simulink model "AGV_Warehouse_Sim_backup_before_v2"  (R2024b)
settings: Solver=ode23t  StartTime=0.0  StopTime=90  MaxStep=0.005  RelTol=1e-3
model workspace: external: MATLAB File D:\agv_robot_matlab\AGV_DataFile.m (data not in the file)
undefined symbols (not defined in the file or in its folder): smiData, X, Y, Z
libraries: sm_lib x478, nesl_utility x11
(part 8 of 8)

== system AGV_Warehouse_Sim_backup_before_v2/AGV_STEP_1_RIGID/Drive_Wheel_Assembly_STEP_4_RIGID/Shaft_Coupling_STEP_1_RIGID ==
  ReferenceFrame : sm_lib/Frames and Transforms/Reference Frame
  Solid : sm_lib/Body Elements/File Solid  ExtGeomFileName=Shaft Coupling.STEP_Default_sldprt.STEP  UnitType=FromFile  ExtGeomFileUnits=m  StepReaderType=HEX  ExportConvexHullGeometry=off  InertiaType=Custom  BasedOnType=DensityFromFile  Density=1000  DensityUnits=kg/m^3  Mass=smiData.Solid(10).mass  MassUnits=kg  CenterOfMass=smiData.Solid(10).CoM  CenterOfMassUnits=m  MomentsOfInertia=smiData.Solid(10).MoI  MomentsOfInertiaUnits=kg*m^2  ProductsOfInertia=smiData.Solid(10).PoI  ProductsOfInertiaUnits=kg*m^2  GraphicType=FromGeometry  MarkerShape=Sphere  MarkerSize=10  GraphicVisPropType=SimpleVisualProperties  GraphicDiffuseColor=smiData.Solid(10).color  GraphicOpacity=smiData.Solid(10).opacity  GraphicSpecularColor=[0.5 0.5 0.5 1.0]  GraphicAmbientColor=[0.15 0.15 0.15 1.0]  GraphicEmissiveColor=[0.0 0.0 0.0 1.0]  GraphicShininess=75  DoExposeReferenceFrame=on  SerializedFrames=<Frames/>
  F : PMIOPort  Side=Left
  connections:
  Solid/RConn1 -- ReferenceFrame/RConn1 -- F/RConn1

== system AGV_Warehouse_Sim_backup_before_v2/AGV_STEP_1_RIGID/Drive_Wheel_Assembly_STEP_4_RIGID/Wheel_Attachment_Bracket_STEP_1_RIGID ==
  ReferenceFrame : sm_lib/Frames and Transforms/Reference Frame
  Solid : sm_lib/Body Elements/File Solid  ExtGeomFileName=Wheel Attachment Bracket.STEP_Default_sldprt.STEP  UnitType=FromFile  ExtGeomFileUnits=m  StepReaderType=HEX  ExportConvexHullGeometry=off  InertiaType=Custom  BasedOnType=DensityFromFile  Density=1000  DensityUnits=kg/m^3  Mass=smiData.Solid(5).mass  MassUnits=kg  CenterOfMass=smiData.Solid(5).CoM  CenterOfMassUnits=m  MomentsOfInertia=smiData.Solid(5).MoI  MomentsOfInertiaUnits=kg*m^2  ProductsOfInertia=smiData.Solid(5).PoI  ProductsOfInertiaUnits=kg*m^2  GraphicType=FromGeometry  MarkerShape=Sphere  MarkerSize=10  GraphicVisPropType=SimpleVisualProperties  GraphicDiffuseColor=smiData.Solid(5).color  GraphicOpacity=smiData.Solid(5).opacity  GraphicSpecularColor=[0.5 0.5 0.5 1.0]  GraphicAmbientColor=[0.15 0.15 0.15 1.0]  GraphicEmissiveColor=[0.0 0.0 0.0 1.0]  GraphicShininess=75  DoExposeReferenceFrame=on  SerializedFrames=<Frames/>
  F : PMIOPort  Side=Left
  connections:
  Solid/RConn1 -- ReferenceFrame/RConn1 -- F/RConn1

== system AGV_Warehouse_Sim_backup_before_v2/AGV_STEP_1_RIGID/Drive_Wheel_Assembly_STEP_4_RIGID/Wheel_Mount_STEP_1_RIGID ==
  ReferenceFrame : sm_lib/Frames and Transforms/Reference Frame
  Solid : sm_lib/Body Elements/File Solid  ExtGeomFileName=Wheel Mount.STEP_Default_sldprt.STEP  UnitType=FromFile  ExtGeomFileUnits=m  StepReaderType=HEX  ExportConvexHullGeometry=off  InertiaType=Custom  BasedOnType=DensityFromFile  Density=1000  DensityUnits=kg/m^3  Mass=smiData.Solid(8).mass  MassUnits=kg  CenterOfMass=smiData.Solid(8).CoM  CenterOfMassUnits=m  MomentsOfInertia=smiData.Solid(8).MoI  MomentsOfInertiaUnits=kg*m^2  ProductsOfInertia=smiData.Solid(8).PoI  ProductsOfInertiaUnits=kg*m^2  GraphicType=FromGeometry  MarkerShape=Sphere  MarkerSize=10  GraphicVisPropType=SimpleVisualProperties  GraphicDiffuseColor=smiData.Solid(8).color  GraphicOpacity=smiData.Solid(8).opacity  GraphicSpecularColor=[0.5 0.5 0.5 1.0]  GraphicAmbientColor=[0.15 0.15 0.15 1.0]  GraphicEmissiveColor=[0.0 0.0 0.0 1.0]  GraphicShininess=75  DoExposeReferenceFrame=on  SerializedFrames=<Frames/>
  F : PMIOPort  Side=Left
  connections:
  Solid/RConn1 -- ReferenceFrame/RConn1 -- F/RConn1

== system AGV_Warehouse_Sim_backup_before_v2/AGV_STEP_1_RIGID/Drive_Wheel_Assembly_STEP_4_RIGID/radial_ball_bearing_68_skf_SKF_61804_18SINC18_68_STEP_1_RIGID ==
  ReferenceFrame : sm_lib/Frames and Transforms/Reference Frame
  Solid : sm_lib/Body Elements/File Solid  ExtGeomFileName=radial ball bearing_68_skf_SKF - 61804 - 18-SI-NC-18_68.STEP_Default_sldprt.STEP  UnitType=FromFile  ExtGeomFileUnits=m  StepReaderType=HEX  ExportConvexHullGeometry=off  InertiaType=Custom  BasedOnType=DensityFromFile  Density=1000  DensityUnits=kg/m^3  Mass=smiData.Solid(6).mass  MassUnits=kg  CenterOfMass=smiData.Solid(6).CoM  CenterOfMassUnits=m  MomentsOfInertia=smiData.Solid(6).MoI  MomentsOfInertiaUnits=kg*m^2  ProductsOfInertia=smiData.Solid(6).PoI  ProductsOfInertiaUnits=kg*m^2  GraphicType=FromGeometry  MarkerShape=Sphere  MarkerSize=10  GraphicVisPropType=SimpleVisualProperties  GraphicDiffuseColor=smiData.Solid(6).color  GraphicOpacity=smiData.Solid(6).opacity  GraphicSpecularColor=[0.5 0.5 0.5 1.0]  GraphicAmbientColor=[0.15 0.15 0.15 1.0]  GraphicEmissiveColor=[0.0 0.0 0.0 1.0]  GraphicShininess=75  DoExposeReferenceFrame=on  SerializedFrames=<Frames/>
  F : PMIOPort  Side=Left
  connections:
  Solid/RConn1 -- ReferenceFrame/RConn1 -- F/RConn1

== system AGV_Warehouse_Sim_backup_before_v2/AGV_STEP_1_RIGID/Front_Back_Casing_Weldment_STEP_1_RIGID/Front_Back_Casing_STEP_1_RIGID ==
  ReferenceFrame : sm_lib/Frames and Transforms/Reference Frame
  Solid : sm_lib/Body Elements/File Solid  ExtGeomFileName=Front Back Casing.STEP_Default_sldprt.STEP  UnitType=FromFile  ExtGeomFileUnits=m  StepReaderType=HEX  ExportConvexHullGeometry=off  InertiaType=Custom  BasedOnType=DensityFromFile  Density=1000  DensityUnits=kg/m^3  Mass=smiData.Solid(22).mass  MassUnits=kg  CenterOfMass=smiData.Solid(22).CoM  CenterOfMassUnits=m  MomentsOfInertia=smiData.Solid(22).MoI  MomentsOfInertiaUnits=kg*m^2  ProductsOfInertia=smiData.Solid(22).PoI  ProductsOfInertiaUnits=kg*m^2  GraphicType=FromGeometry  MarkerShape=Sphere  MarkerSize=10  GraphicVisPropType=SimpleVisualProperties  GraphicDiffuseColor=smiData.Solid(22).color  GraphicOpacity=smiData.Solid(22).opacity  GraphicSpecularColor=[0.5 0.5 0.5 1.0]  GraphicAmbientColor=[0.15 0.15 0.15 1.0]  GraphicEmissiveColor=[0.0 0.0 0.0 1.0]  GraphicShininess=75  DoExposeReferenceFrame=on  SerializedFrames=<Frames/>
  F : PMIOPort  Side=Left
  connections:
  Solid/RConn1 -- ReferenceFrame/RConn1 -- F/RConn1

== system AGV_Warehouse_Sim_backup_before_v2/AGV_STEP_1_RIGID/Front_Back_Casing_Weldment_STEP_1_RIGID/hex_nut_style_1_gradeab_iso_ISO_4032_M4_W_N_STEP_10_RIGID ==
  ReferenceFrame : sm_lib/Frames and Transforms/Reference Frame
  Solid : sm_lib/Body Elements/File Solid  ExtGeomFileName=hex nut style 1 gradeab_iso_ISO - 4032 - M4 - W - N.STEP_Default_sldprt.STEP  UnitType=FromFile  ExtGeomFileUnits=m  StepReaderType=HEX  ExportConvexHullGeometry=off  InertiaType=Custom  BasedOnType=DensityFromFile  Density=1000  DensityUnits=kg/m^3  Mass=smiData.Solid(21).mass  MassUnits=kg  CenterOfMass=smiData.Solid(21).CoM  CenterOfMassUnits=m  MomentsOfInertia=smiData.Solid(21).MoI  MomentsOfInertiaUnits=kg*m^2  ProductsOfInertia=smiData.Solid(21).PoI  ProductsOfInertiaUnits=kg*m^2  GraphicType=FromGeometry  MarkerShape=Sphere  MarkerSize=10  GraphicVisPropType=SimpleVisualProperties  GraphicDiffuseColor=smiData.Solid(21).color  GraphicOpacity=smiData.Solid(21).opacity  GraphicSpecularColor=[0.5 0.5 0.5 1.0]  GraphicAmbientColor=[0.15 0.15 0.15 1.0]  GraphicEmissiveColor=[0.0 0.0 0.0 1.0]  GraphicShininess=75  DoExposeReferenceFrame=on  SerializedFrames=<Frames/>
  F : PMIOPort  Side=Left
  connections:
  Solid/RConn1 -- ReferenceFrame/RConn1 -- F/RConn1

== system AGV_Warehouse_Sim_backup_before_v2/AGV_STEP_1_RIGID/Front_Back_Casing_Weldment_STEP_1_RIGID/hex_nut_style_1_gradeab_iso_ISO_4032_M4_W_N_STEP_11_RIGID ==
  ReferenceFrame : sm_lib/Frames and Transforms/Reference Frame
  Solid : sm_lib/Body Elements/File Solid  ExtGeomFileName=hex nut style 1 gradeab_iso_ISO - 4032 - M4 - W - N.STEP_Default_sldprt.STEP  UnitType=FromFile  ExtGeomFileUnits=m  StepReaderType=HEX  ExportConvexHullGeometry=off  InertiaType=Custom  BasedOnType=DensityFromFile  Density=1000  DensityUnits=kg/m^3  Mass=smiData.Solid(21).mass  MassUnits=kg  CenterOfMass=smiData.Solid(21).CoM  CenterOfMassUnits=m  MomentsOfInertia=smiData.Solid(21).MoI  MomentsOfInertiaUnits=kg*m^2  ProductsOfInertia=smiData.Solid(21).PoI  ProductsOfInertiaUnits=kg*m^2  GraphicType=FromGeometry  MarkerShape=Sphere  MarkerSize=10  GraphicVisPropType=SimpleVisualProperties  GraphicDiffuseColor=smiData.Solid(21).color  GraphicOpacity=smiData.Solid(21).opacity  GraphicSpecularColor=[0.5 0.5 0.5 1.0]  GraphicAmbientColor=[0.15 0.15 0.15 1.0]  GraphicEmissiveColor=[0.0 0.0 0.0 1.0]  GraphicShininess=75  DoExposeReferenceFrame=on  SerializedFrames=<Frames/>
  F : PMIOPort  Side=Left
  connections:
  Solid/RConn1 -- ReferenceFrame/RConn1 -- F/RConn1

== system AGV_Warehouse_Sim_backup_before_v2/AGV_STEP_1_RIGID/Front_Back_Casing_Weldment_STEP_1_RIGID/hex_nut_style_1_gradeab_iso_ISO_4032_M4_W_N_STEP_12_RIGID ==
  ReferenceFrame : sm_lib/Frames and Transforms/Reference Frame
  Solid : sm_lib/Body Elements/File Solid  ExtGeomFileName=hex nut style 1 gradeab_iso_ISO - 4032 - M4 - W - N.STEP_Default_sldprt.STEP  UnitType=FromFile  ExtGeomFileUnits=m  StepReaderType=HEX  ExportConvexHullGeometry=off  InertiaType=Custom  BasedOnType=DensityFromFile  Density=1000  DensityUnits=kg/m^3  Mass=smiData.Solid(21).mass  MassUnits=kg  CenterOfMass=smiData.Solid(21).CoM  CenterOfMassUnits=m  MomentsOfInertia=smiData.Solid(21).MoI  MomentsOfInertiaUnits=kg*m^2  ProductsOfInertia=smiData.Solid(21).PoI  ProductsOfInertiaUnits=kg*m^2  GraphicType=FromGeometry  MarkerShape=Sphere  MarkerSize=10  GraphicVisPropType=SimpleVisualProperties  GraphicDiffuseColor=smiData.Solid(21).color  GraphicOpacity=smiData.Solid(21).opacity  GraphicSpecularColor=[0.5 0.5 0.5 1.0]  GraphicAmbientColor=[0.15 0.15 0.15 1.0]  GraphicEmissiveColor=[0.0 0.0 0.0 1.0]  GraphicShininess=75  DoExposeReferenceFrame=on  SerializedFrames=<Frames/>
  F : PMIOPort  Side=Left
  connections:
  Solid/RConn1 -- ReferenceFrame/RConn1 -- F/RConn1

== system AGV_Warehouse_Sim_backup_before_v2/AGV_STEP_1_RIGID/Front_Back_Casing_Weldment_STEP_1_RIGID/hex_nut_style_1_gradeab_iso_ISO_4032_M4_W_N_STEP_13_RIGID ==
  ReferenceFrame : sm_lib/Frames and Transforms/Reference Frame
  Solid : sm_lib/Body Elements/File Solid  ExtGeomFileName=hex nut style 1 gradeab_iso_ISO - 4032 - M4 - W - N.STEP_Default_sldprt.STEP  UnitType=FromFile  ExtGeomFileUnits=m  StepReaderType=HEX  ExportConvexHullGeometry=off  InertiaType=Custom  BasedOnType=DensityFromFile  Density=1000  DensityUnits=kg/m^3  Mass=smiData.Solid(21).mass  MassUnits=kg  CenterOfMass=smiData.Solid(21).CoM  CenterOfMassUnits=m  MomentsOfInertia=smiData.Solid(21).MoI  MomentsOfInertiaUnits=kg*m^2  ProductsOfInertia=smiData.Solid(21).PoI  ProductsOfInertiaUnits=kg*m^2  GraphicType=FromGeometry  MarkerShape=Sphere  MarkerSize=10  GraphicVisPropType=SimpleVisualProperties  GraphicDiffuseColor=smiData.Solid(21).color  GraphicOpacity=smiData.Solid(21).opacity  GraphicSpecularColor=[0.5 0.5 0.5 1.0]  GraphicAmbientColor=[0.15 0.15 0.15 1.0]  GraphicEmissiveColor=[0.0 0.0 0.0 1.0]  GraphicShininess=75  DoExposeReferenceFrame=on  SerializedFrames=<Frames/>
  F : PMIOPort  Side=Left
  connections:
  Solid/RConn1 -- ReferenceFrame/RConn1 -- F/RConn1

== system AGV_Warehouse_Sim_backup_before_v2/AGV_STEP_1_RIGID/Front_Back_Casing_Weldment_STEP_1_RIGID/hex_nut_style_1_gradeab_iso_ISO_4032_M4_W_N_STEP_14_RIGID ==
  ReferenceFrame : sm_lib/Frames and Transforms/Reference Frame
  Solid : sm_lib/Body Elements/File Solid  ExtGeomFileName=hex nut style 1 gradeab_iso_ISO - 4032 - M4 - W - N.STEP_Default_sldprt.STEP  UnitType=FromFile  ExtGeomFileUnits=m  StepReaderType=HEX  ExportConvexHullGeometry=off  InertiaType=Custom  BasedOnType=DensityFromFile  Density=1000  DensityUnits=kg/m^3  Mass=smiData.Solid(21).mass  MassUnits=kg  CenterOfMass=smiData.Solid(21).CoM  CenterOfMassUnits=m  MomentsOfInertia=smiData.Solid(21).MoI  MomentsOfInertiaUnits=kg*m^2  ProductsOfInertia=smiData.Solid(21).PoI  ProductsOfInertiaUnits=kg*m^2  GraphicType=FromGeometry  MarkerShape=Sphere  MarkerSize=10  GraphicVisPropType=SimpleVisualProperties  GraphicDiffuseColor=smiData.Solid(21).color  GraphicOpacity=smiData.Solid(21).opacity  GraphicSpecularColor=[0.5 0.5 0.5 1.0]  GraphicAmbientColor=[0.15 0.15 0.15 1.0]  GraphicEmissiveColor=[0.0 0.0 0.0 1.0]  GraphicShininess=75  DoExposeReferenceFrame=on  SerializedFrames=<Frames/>
  F : PMIOPort  Side=Left
  connections:
  Solid/RConn1 -- ReferenceFrame/RConn1 -- F/RConn1

== system AGV_Warehouse_Sim_backup_before_v2/AGV_STEP_1_RIGID/Front_Back_Casing_Weldment_STEP_1_RIGID/hex_nut_style_1_gradeab_iso_ISO_4032_M4_W_N_STEP_1_RIGID ==
  ReferenceFrame : sm_lib/Frames and Transforms/Reference Frame
  Solid : sm_lib/Body Elements/File Solid  ExtGeomFileName=hex nut style 1 gradeab_iso_ISO - 4032 - M4 - W - N.STEP_Default_sldprt.STEP  UnitType=FromFile  ExtGeomFileUnits=m  StepReaderType=HEX  ExportConvexHullGeometry=off  InertiaType=Custom  BasedOnType=DensityFromFile  Density=1000  DensityUnits=kg/m^3  Mass=smiData.Solid(21).mass  MassUnits=kg  CenterOfMass=smiData.Solid(21).CoM  CenterOfMassUnits=m  MomentsOfInertia=smiData.Solid(21).MoI  MomentsOfInertiaUnits=kg*m^2  ProductsOfInertia=smiData.Solid(21).PoI  ProductsOfInertiaUnits=kg*m^2  GraphicType=FromGeometry  MarkerShape=Sphere  MarkerSize=10  GraphicVisPropType=SimpleVisualProperties  GraphicDiffuseColor=smiData.Solid(21).color  GraphicOpacity=smiData.Solid(21).opacity  GraphicSpecularColor=[0.5 0.5 0.5 1.0]  GraphicAmbientColor=[0.15 0.15 0.15 1.0]  GraphicEmissiveColor=[0.0 0.0 0.0 1.0]  GraphicShininess=75  DoExposeReferenceFrame=on  SerializedFrames=<Frames/>
  F : PMIOPort  Side=Left
  connections:
  Solid/RConn1 -- ReferenceFrame/RConn1 -- F/RConn1

== system AGV_Warehouse_Sim_backup_before_v2/AGV_STEP_1_RIGID/Front_Back_Casing_Weldment_STEP_1_RIGID/hex_nut_style_1_gradeab_iso_ISO_4032_M4_W_N_STEP_2_RIGID ==
  ReferenceFrame : sm_lib/Frames and Transforms/Reference Frame
  Solid : sm_lib/Body Elements/File Solid  ExtGeomFileName=hex nut style 1 gradeab_iso_ISO - 4032 - M4 - W - N.STEP_Default_sldprt.STEP  UnitType=FromFile  ExtGeomFileUnits=m  StepReaderType=HEX  ExportConvexHullGeometry=off  InertiaType=Custom  BasedOnType=DensityFromFile  Density=1000  DensityUnits=kg/m^3  Mass=smiData.Solid(21).mass  MassUnits=kg  CenterOfMass=smiData.Solid(21).CoM  CenterOfMassUnits=m  MomentsOfInertia=smiData.Solid(21).MoI  MomentsOfInertiaUnits=kg*m^2  ProductsOfInertia=smiData.Solid(21).PoI  ProductsOfInertiaUnits=kg*m^2  GraphicType=FromGeometry  MarkerShape=Sphere  MarkerSize=10  GraphicVisPropType=SimpleVisualProperties  GraphicDiffuseColor=smiData.Solid(21).color  GraphicOpacity=smiData.Solid(21).opacity  GraphicSpecularColor=[0.5 0.5 0.5 1.0]  GraphicAmbientColor=[0.15 0.15 0.15 1.0]  GraphicEmissiveColor=[0.0 0.0 0.0 1.0]  GraphicShininess=75  DoExposeReferenceFrame=on  SerializedFrames=<Frames/>
  F : PMIOPort  Side=Left
  connections:
  Solid/RConn1 -- ReferenceFrame/RConn1 -- F/RConn1

== system AGV_Warehouse_Sim_backup_before_v2/AGV_STEP_1_RIGID/Front_Back_Casing_Weldment_STEP_1_RIGID/hex_nut_style_1_gradeab_iso_ISO_4032_M4_W_N_STEP_3_RIGID ==
  ReferenceFrame : sm_lib/Frames and Transforms/Reference Frame
  Solid : sm_lib/Body Elements/File Solid  ExtGeomFileName=hex nut style 1 gradeab_iso_ISO - 4032 - M4 - W - N.STEP_Default_sldprt.STEP  UnitType=FromFile  ExtGeomFileUnits=m  StepReaderType=HEX  ExportConvexHullGeometry=off  InertiaType=Custom  BasedOnType=DensityFromFile  Density=1000  DensityUnits=kg/m^3  Mass=smiData.Solid(21).mass  MassUnits=kg  CenterOfMass=smiData.Solid(21).CoM  CenterOfMassUnits=m  MomentsOfInertia=smiData.Solid(21).MoI  MomentsOfInertiaUnits=kg*m^2  ProductsOfInertia=smiData.Solid(21).PoI  ProductsOfInertiaUnits=kg*m^2  GraphicType=FromGeometry  MarkerShape=Sphere  MarkerSize=10  GraphicVisPropType=SimpleVisualProperties  GraphicDiffuseColor=smiData.Solid(21).color  GraphicOpacity=smiData.Solid(21).opacity  GraphicSpecularColor=[0.5 0.5 0.5 1.0]  GraphicAmbientColor=[0.15 0.15 0.15 1.0]  GraphicEmissiveColor=[0.0 0.0 0.0 1.0]  GraphicShininess=75  DoExposeReferenceFrame=on  SerializedFrames=<Frames/>
  F : PMIOPort  Side=Left
  connections:
  Solid/RConn1 -- ReferenceFrame/RConn1 -- F/RConn1

== system AGV_Warehouse_Sim_backup_before_v2/AGV_STEP_1_RIGID/Front_Back_Casing_Weldment_STEP_1_RIGID/hex_nut_style_1_gradeab_iso_ISO_4032_M4_W_N_STEP_4_RIGID ==
  ReferenceFrame : sm_lib/Frames and Transforms/Reference Frame
  Solid : sm_lib/Body Elements/File Solid  ExtGeomFileName=hex nut style 1 gradeab_iso_ISO - 4032 - M4 - W - N.STEP_Default_sldprt.STEP  UnitType=FromFile  ExtGeomFileUnits=m  StepReaderType=HEX  ExportConvexHullGeometry=off  InertiaType=Custom  BasedOnType=DensityFromFile  Density=1000  DensityUnits=kg/m^3  Mass=smiData.Solid(21).mass  MassUnits=kg  CenterOfMass=smiData.Solid(21).CoM  CenterOfMassUnits=m  MomentsOfInertia=smiData.Solid(21).MoI  MomentsOfInertiaUnits=kg*m^2  ProductsOfInertia=smiData.Solid(21).PoI  ProductsOfInertiaUnits=kg*m^2  GraphicType=FromGeometry  MarkerShape=Sphere  MarkerSize=10  GraphicVisPropType=SimpleVisualProperties  GraphicDiffuseColor=smiData.Solid(21).color  GraphicOpacity=smiData.Solid(21).opacity  GraphicSpecularColor=[0.5 0.5 0.5 1.0]  GraphicAmbientColor=[0.15 0.15 0.15 1.0]  GraphicEmissiveColor=[0.0 0.0 0.0 1.0]  GraphicShininess=75  DoExposeReferenceFrame=on  SerializedFrames=<Frames/>
  F : PMIOPort  Side=Left
  connections:
  Solid/RConn1 -- ReferenceFrame/RConn1 -- F/RConn1

== system AGV_Warehouse_Sim_backup_before_v2/AGV_STEP_1_RIGID/Front_Back_Casing_Weldment_STEP_1_RIGID/hex_nut_style_1_gradeab_iso_ISO_4032_M4_W_N_STEP_5_RIGID ==
  ReferenceFrame : sm_lib/Frames and Transforms/Reference Frame
  Solid : sm_lib/Body Elements/File Solid  ExtGeomFileName=hex nut style 1 gradeab_iso_ISO - 4032 - M4 - W - N.STEP_Default_sldprt.STEP  UnitType=FromFile  ExtGeomFileUnits=m  StepReaderType=HEX  ExportConvexHullGeometry=off  InertiaType=Custom  BasedOnType=DensityFromFile  Density=1000  DensityUnits=kg/m^3  Mass=smiData.Solid(21).mass  MassUnits=kg  CenterOfMass=smiData.Solid(21).CoM  CenterOfMassUnits=m  MomentsOfInertia=smiData.Solid(21).MoI  MomentsOfInertiaUnits=kg*m^2  ProductsOfInertia=smiData.Solid(21).PoI  ProductsOfInertiaUnits=kg*m^2  GraphicType=FromGeometry  MarkerShape=Sphere  MarkerSize=10  GraphicVisPropType=SimpleVisualProperties  GraphicDiffuseColor=smiData.Solid(21).color  GraphicOpacity=smiData.Solid(21).opacity  GraphicSpecularColor=[0.5 0.5 0.5 1.0]  GraphicAmbientColor=[0.15 0.15 0.15 1.0]  GraphicEmissiveColor=[0.0 0.0 0.0 1.0]  GraphicShininess=75  DoExposeReferenceFrame=on  SerializedFrames=<Frames/>
  F : PMIOPort  Side=Left
  connections:
  Solid/RConn1 -- ReferenceFrame/RConn1 -- F/RConn1

== system AGV_Warehouse_Sim_backup_before_v2/AGV_STEP_1_RIGID/Front_Back_Casing_Weldment_STEP_1_RIGID/hex_nut_style_1_gradeab_iso_ISO_4032_M4_W_N_STEP_6_RIGID ==
  ReferenceFrame : sm_lib/Frames and Transforms/Reference Frame
  Solid : sm_lib/Body Elements/File Solid  ExtGeomFileName=hex nut style 1 gradeab_iso_ISO - 4032 - M4 - W - N.STEP_Default_sldprt.STEP  UnitType=FromFile  ExtGeomFileUnits=m  StepReaderType=HEX  ExportConvexHullGeometry=off  InertiaType=Custom  BasedOnType=DensityFromFile  Density=1000  DensityUnits=kg/m^3  Mass=smiData.Solid(21).mass  MassUnits=kg  CenterOfMass=smiData.Solid(21).CoM  CenterOfMassUnits=m  MomentsOfInertia=smiData.Solid(21).MoI  MomentsOfInertiaUnits=kg*m^2  ProductsOfInertia=smiData.Solid(21).PoI  ProductsOfInertiaUnits=kg*m^2  GraphicType=FromGeometry  MarkerShape=Sphere  MarkerSize=10  GraphicVisPropType=SimpleVisualProperties  GraphicDiffuseColor=smiData.Solid(21).color  GraphicOpacity=smiData.Solid(21).opacity  GraphicSpecularColor=[0.5 0.5 0.5 1.0]  GraphicAmbientColor=[0.15 0.15 0.15 1.0]  GraphicEmissiveColor=[0.0 0.0 0.0 1.0]  GraphicShininess=75  DoExposeReferenceFrame=on  SerializedFrames=<Frames/>
  F : PMIOPort  Side=Left
  connections:
  Solid/RConn1 -- ReferenceFrame/RConn1 -- F/RConn1

== system AGV_Warehouse_Sim_backup_before_v2/AGV_STEP_1_RIGID/Front_Back_Casing_Weldment_STEP_1_RIGID/hex_nut_style_1_gradeab_iso_ISO_4032_M4_W_N_STEP_7_RIGID ==
  ReferenceFrame : sm_lib/Frames and Transforms/Reference Frame
  Solid : sm_lib/Body Elements/File Solid  ExtGeomFileName=hex nut style 1 gradeab_iso_ISO - 4032 - M4 - W - N.STEP_Default_sldprt.STEP  UnitType=FromFile  ExtGeomFileUnits=m  StepReaderType=HEX  ExportConvexHullGeometry=off  InertiaType=Custom  BasedOnType=DensityFromFile  Density=1000  DensityUnits=kg/m^3  Mass=smiData.Solid(21).mass  MassUnits=kg  CenterOfMass=smiData.Solid(21).CoM  CenterOfMassUnits=m  MomentsOfInertia=smiData.Solid(21).MoI  MomentsOfInertiaUnits=kg*m^2  ProductsOfInertia=smiData.Solid(21).PoI  ProductsOfInertiaUnits=kg*m^2  GraphicType=FromGeometry  MarkerShape=Sphere  MarkerSize=10  GraphicVisPropType=SimpleVisualProperties  GraphicDiffuseColor=smiData.Solid(21).color  GraphicOpacity=smiData.Solid(21).opacity  GraphicSpecularColor=[0.5 0.5 0.5 1.0]  GraphicAmbientColor=[0.15 0.15 0.15 1.0]  GraphicEmissiveColor=[0.0 0.0 0.0 1.0]  GraphicShininess=75  DoExposeReferenceFrame=on  SerializedFrames=<Frames/>
  F : PMIOPort  Side=Left
  connections:
  Solid/RConn1 -- ReferenceFrame/RConn1 -- F/RConn1

== system AGV_Warehouse_Sim_backup_before_v2/AGV_STEP_1_RIGID/Front_Back_Casing_Weldment_STEP_1_RIGID/hex_nut_style_1_gradeab_iso_ISO_4032_M4_W_N_STEP_8_RIGID ==
  ReferenceFrame : sm_lib/Frames and Transforms/Reference Frame
  Solid : sm_lib/Body Elements/File Solid  ExtGeomFileName=hex nut style 1 gradeab_iso_ISO - 4032 - M4 - W - N.STEP_Default_sldprt.STEP  UnitType=FromFile  ExtGeomFileUnits=m  StepReaderType=HEX  ExportConvexHullGeometry=off  InertiaType=Custom  BasedOnType=DensityFromFile  Density=1000  DensityUnits=kg/m^3  Mass=smiData.Solid(21).mass  MassUnits=kg  CenterOfMass=smiData.Solid(21).CoM  CenterOfMassUnits=m  MomentsOfInertia=smiData.Solid(21).MoI  MomentsOfInertiaUnits=kg*m^2  ProductsOfInertia=smiData.Solid(21).PoI  ProductsOfInertiaUnits=kg*m^2  GraphicType=FromGeometry  MarkerShape=Sphere  MarkerSize=10  GraphicVisPropType=SimpleVisualProperties  GraphicDiffuseColor=smiData.Solid(21).color  GraphicOpacity=smiData.Solid(21).opacity  GraphicSpecularColor=[0.5 0.5 0.5 1.0]  GraphicAmbientColor=[0.15 0.15 0.15 1.0]  GraphicEmissiveColor=[0.0 0.0 0.0 1.0]  GraphicShininess=75  DoExposeReferenceFrame=on  SerializedFrames=<Frames/>
  F : PMIOPort  Side=Left
  connections:
  Solid/RConn1 -- ReferenceFrame/RConn1 -- F/RConn1

== system AGV_Warehouse_Sim_backup_before_v2/AGV_STEP_1_RIGID/Front_Back_Casing_Weldment_STEP_1_RIGID/hex_nut_style_1_gradeab_iso_ISO_4032_M4_W_N_STEP_9_RIGID ==
  ReferenceFrame : sm_lib/Frames and Transforms/Reference Frame
  Solid : sm_lib/Body Elements/File Solid  ExtGeomFileName=hex nut style 1 gradeab_iso_ISO - 4032 - M4 - W - N.STEP_Default_sldprt.STEP  UnitType=FromFile  ExtGeomFileUnits=m  StepReaderType=HEX  ExportConvexHullGeometry=off  InertiaType=Custom  BasedOnType=DensityFromFile  Density=1000  DensityUnits=kg/m^3  Mass=smiData.Solid(21).mass  MassUnits=kg  CenterOfMass=smiData.Solid(21).CoM  CenterOfMassUnits=m  MomentsOfInertia=smiData.Solid(21).MoI  MomentsOfInertiaUnits=kg*m^2  ProductsOfInertia=smiData.Solid(21).PoI  ProductsOfInertiaUnits=kg*m^2  GraphicType=FromGeometry  MarkerShape=Sphere  MarkerSize=10  GraphicVisPropType=SimpleVisualProperties  GraphicDiffuseColor=smiData.Solid(21).color  GraphicOpacity=smiData.Solid(21).opacity  GraphicSpecularColor=[0.5 0.5 0.5 1.0]  GraphicAmbientColor=[0.15 0.15 0.15 1.0]  GraphicEmissiveColor=[0.0 0.0 0.0 1.0]  GraphicShininess=75  DoExposeReferenceFrame=on  SerializedFrames=<Frames/>
  F : PMIOPort  Side=Left
  connections:
  Solid/RConn1 -- ReferenceFrame/RConn1 -- F/RConn1

== matlab function AGV_Warehouse_Sim_backup_before_v2/Line_Tracking_Controller ==
  settings: updateMethod=DISCRETE  sampleTime=0.01
  data: pos input; tau_L output; yaw input; t input; tau_R output; e_lat output; e_heading output; state_out output; station_out output
function [tau_L, tau_R, e_lat, e_heading, state_out, station_out] = Line_Tracking_Controller(pos, yaw, t)
% AGV Line-Tracking, Along-Track Corner Capture, Rate-Limited Torque Control
% pos: [X, Y] in meters (World frame)
% yaw: chassis orientation in radians (World frame)
% t: simulation time in seconds

X = pos(1);
Y = pos(2);

% 3 Exact Pallet Station Waypoints projected onto the black track loop:
% Blue Station:  (0.0, -3.0)
% Green Station: (5.0,  0.0)
% Red Station:   (-2.5, 3.0)
stations = [  0.0, -3.0; ...  % 1: Blue Station
              5.0,  0.0; ...  % 2: Green Station
             -2.5,  3.0 ];    % 3: Red Station

% 4 Track Edges (Start -> End vertices along the rectangular loop):
% Edge 1 (South): (-5.0, -3.0) -> ( 5.0, -3.0)  Heading:  0.0 rad (  0 deg)
% Edge 2 (East):  ( 5.0, -3.0) -> ( 5.0,  3.0)  Heading:  pi/2 rad (+90 deg)
% Edge 3 (North): ( 5.0,  3.0) -> (-5.0,  3.0)  Heading:  pi rad   (180 deg)
% Edge 4 (West):  (-5.0,  3.0) -> (-5.0, -3.0)  Heading: -pi/2 rad (-90 deg)
edge_starts = [-5.0, -3.0; ...
                5.0, -3.0; ...
                5.0,  3.0; ...
               -5.0,  3.0];
edge_ends   = [ 5.0, -3.0; ...
                5.0,  3.0; ...
               -5.0,  3.0; ...
               -5.0, -3.0];

yaw_des_table = [0.0, pi/2, pi, -pi/2];

% State Machine States:
% 0: FOLLOW_STRAIGHT
% 1: STOP_AT_PALLET
% 2: PIVOT_CORNER
% 3: COOLDOWN_PALLET
persistent state target_station t_stop_start t_cooldown_start
persistent current_edge theta_prev X_prev Y_prev e_int_L e_int_R
persistent tau_L_prev tau_R_prev

if isempty(state)
    state = 0;
    target_station = 1;
    t_stop_start = 0.0;
    t_cooldown_start = 0.0;
    current_edge = 1;
    theta_prev = atan2(-sin(yaw), -cos(yaw));
    X_prev = X;
    Y_prev = Y;
    e_int_L = 0.0;
    e_int_R = 0.0;
    tau_L_prev = 0.0;
    tau_R_prev = 0.0;
end

% Kinematic Calculations (Sample Time dt = 0.01 s)
dt = 0.01;
% Navigation heading theta (where 0 rad = +X, pi/2 = +Y, pi = -X, -pi/2 = -Y)
theta = atan2(-sin(yaw), -cos(yaw));

% Chassis Angular Velocity wz (rad/s) with phase-wrap protection:
dtheta = atan2(sin(theta - theta_prev), cos(theta - theta_prev));
wz = dtheta / dt;
theta_prev = theta;

% Forward chassis velocity:
vx = (X - X_prev) / dt;
vy = (Y - Y_prev) / dt;
v_fwd_meas = vx * cos(theta) + vy * sin(theta);
X_prev = X;
Y_prev = Y;

R_wheel = 0.073182;  % Wheel outer radius (m)
b_track = 0.629;     % Half track width (m) [W = 1.258 m]

% Actual wheel speeds from chassis kinematics (rad/s):
w_L_act = (v_fwd_meas - wz * b_track) / R_wheel;
w_R_act = (v_fwd_meas + wz * b_track) / R_wheel;

% Target Heading and Cross-Track Lateral Error for Current Edge
yaw_des = yaw_des_table(current_edge);
e_yaw = atan2(sin(yaw_des - theta), cos(yaw_des - theta));

if current_edge == 1 % South edge (Y = -3.0, moving +X)
    e_lat = -3.0 - Y;
elseif current_edge == 2 % East edge (X = 5.0, moving +Y)
    e_lat = X - 5.0;
elseif current_edge == 3 % North edge (Y = 3.0, moving -X)
    e_lat = Y - 3.0;
else % West edge (X = -5.0, moving -Y)
    e_lat = -5.0 - X;
end

% Along-Track Scalar Projection to Next Corner Vertex
P_curr = edge_starts(current_edge, :)';
P_next = edge_ends(current_edge, :)';
seg_vec = P_next - P_curr;
u_seg = seg_vec / norm(seg_vec);
along_dist_to_corner = dot(P_next - [X; Y], u_seg);

% Pallet Station Proximity (within 0.20 m of target bay)
P_tgt = stations(target_station, :)';
dist_station = norm([X; Y] - P_tgt);

% State Transitions
if state == 0 % FOLLOW_STRAIGHT
    if dist_station < 0.20
        state = 1; % Enter STOP_AT_PALLET
        t_stop_start = t;
    elseif along_dist_to_corner <= 0.12
        current_edge = mod(current_edge, 4) + 1; % Advance to next track edge
        state = 2; % Enter PIVOT_CORNER
    end
elseif state == 1 % STOP_AT_PALLET (3.0-second full stop)
    if (t - t_stop_start) >= 3.0
        state = 3; % Enter COOLDOWN_PALLET
        t_cooldown_start = t;
        target_station = mod(target_station, 3) + 1; % Next pallet bay
    end
elseif state == 2 % PIVOT_CORNER (v_fwd = 0 until abs(e_yaw) < 0.05 rad)
    yaw_des_corner = yaw_des_table(current_edge);
    e_yaw_corner = atan2(sin(yaw_des_corner - theta), cos(yaw_des_corner - theta));
    if abs(e_yaw_corner) < 0.05 % Reached within ~2.86 degrees of perpendicular heading
        state = 0; % Switch back to FOLLOW_STRAIGHT
    end
elseif state == 3 % COOLDOWN_PALLET (lockout for 3.0 s, but corner capture active)
    if along_dist_to_corner <= 0.12
        current_edge = mod(current_edge, 4) + 1;
        state = 2; % Enter PIVOT_CORNER
    elseif (t - t_cooldown_start) >= 3.0
        state = 0; % Cooldown finished, resume normal tracking
    end
end

% Target Wheel Commands / Direct Torque Calculation
w_base = 0.35 / R_wheel; % Base cruise wheel speed (~4.78 rad/s)

if state == 1 % STOP_AT_PALLET: target zero speed
    w_L_cmd = 0.0;
    w_R_cmd = 0.0;
    err_L = w_L_cmd - w_L_act;
    err_R = w_R_cmd - w_R_act;
    e_int_L = e_int_L + err_L * dt;
    e_int_R = e_int_R + err_R * dt;
    e_int_L = max(-1.0, min(1.0, e_int_L));
    e_int_R = max(-1.0, min(1.0, e_int_R));
    tau_L_target = 2.0 * err_L + 0.5 * e_int_L;
    tau_R_target = 2.0 * err_R + 0.5 * e_int_R;
elseif state == 2 % PIVOT_CORNER: pure counter-rotating pivot at v_fwd = 0
    yaw_des_corner = yaw_des_table(current_edge);
    e_yaw_corner = atan2(sin(yaw_des_corner - theta), cos(yaw_des_corner - theta));
    s_yaw = sign(e_yaw_corner);
    if s_yaw == 0, s_yaw = 1.0; end
    w_L_cmd = -s_yaw * 1.8;
    w_R_cmd = +s_yaw * 1.8;
    err_L = w_L_cmd - w_L_act;
    err_R = w_R_cmd - w_R_act;
    tau_L_target = 1.5 * err_L;
    tau_R_target = 1.5 * err_R;
else % FOLLOW_STRAIGHT (0) or COOLDOWN_PALLET (3)
    Kp_lat = 2.0;
    Kp_yaw = 1.5;
    Kd_yaw = 0.3;
    w_diff = Kp_lat * e_lat + Kp_yaw * e_yaw - Kd_yaw * wz;
    w_L_cmd = w_base - w_diff;
    w_R_cmd = w_base + w_diff;
    err_L = w_L_cmd - w_L_act;
    err_R = w_R_cmd - w_R_act;
    e_int_L = e_int_L + err_L * dt;
    e_int_R = e_int_R + err_R * dt;
    e_int_L = max(-1.0, min(1.0, e_int_L));
    e_int_R = max(-1.0, min(1.0, e_int_R));
    tau_L_target = 2.0 * err_L + 0.3 * e_int_L;
    tau_R_target = 2.0 * err_R + 0.3 * e_int_R;
end

% Smooth Output Ramping (max slew = 3.0 N*m/s => delta_tau_max = 0.03 N*m per 0.01 s step)
delta_tau_max = 3.0 * dt;
tau_L_ramped = tau_L_prev + max(-delta_tau_max, min(delta_tau_max, tau_L_target - tau_L_prev));
tau_R_ramped = tau_R_prev + max(-delta_tau_max, min(delta_tau_max, tau_R_target - tau_R_prev));
tau_L_prev = tau_L_ramped;
tau_R_prev = tau_R_ramped;

% Strict Torque Saturation ([-1.2, +1.2] N*m)
tau_limit = 1.2;
tau_L = max(-tau_limit, min(tau_limit, tau_L_ramped));
tau_R = max(-tau_limit, min(tau_limit, tau_R_ramped));

state_out = double(state);
station_out = double(target_station);
e_heading = e_yaw;
